simulink model "cartpole_pulse"  (R2024b)
settings: Solver=ode45  StartTime=0.0  StopTime=8  MaxStep=0.001  RelTol=1e-10  AbsTol=1e-12
model workspace (MAT data in the model file):
  A = [0  1  0  0; 0  -0.181818181818  2.67545454545  0; 0  0  0  1; 0  -0.454545454545  31.2136363636  0]
  B = [0; 1.81818181818; 0; 4.54545454545]
  K = [-38.7298334621 -36.3830062182 160.925764173 29.6787056292]
  pulse_amplitude = 2
  x0 = [0; 0; 0; 0]
Description:
  | Undergraduate thesis reimplementation. State=[x v theta omega], SI units; xc=x-l*sin(theta). Model Workspace contains exact Table 1 parameters and baseline A controller.
settings Model: ModifiedByFormat=WANG Zheng  Creator=WANG Zheng  LastModifiedBy=WANG Zheng
settings DataIOCC: OutputOption=SpecifiedOutputTimes  OutputTimes=[0:0.001:8]

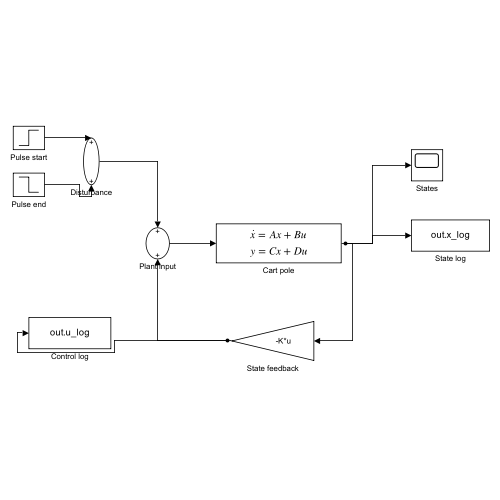
[thumbnail: Simulink's stored preview of the top-level diagram]
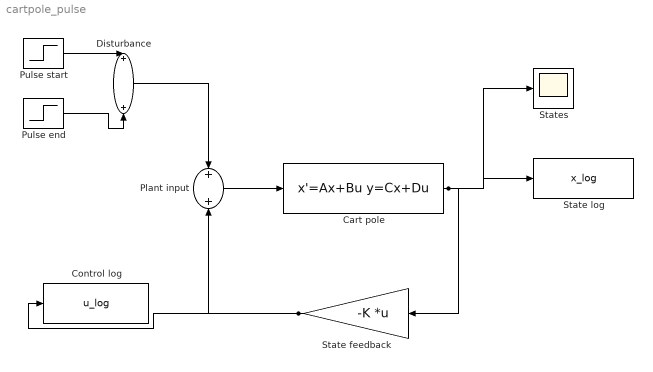
== system cartpole_pulse ==
  Cart pole : StateSpace  A=A  B=B  C=eye(4)  D=zeros(4,1)  InitialCondition=x0
  Control log : ToWorkspace  VariableName=u_log  SaveFormat=Timeseries  SampleTime=-1
  Disturbance : Sum
  Plant input : Sum
  Pulse end : Step  Time=1.2  After=-pulse_amplitude  SampleTime=0
  Pulse start : Step  After=pulse_amplitude  SampleTime=0
  State feedback : Gain  Gain=-K  Multiplication=Matrix(K*u)
  State log : ToWorkspace  VariableName=x_log  SaveFormat=Timeseries  SampleTime=-1
  States : Scope
  wires:
  Pulse start/1 -> Disturbance/1
  Pulse end/1 -> Disturbance/2
  Disturbance/1 -> Plant input/1
  State feedback/1 -> Plant input/2, Control log/1
  Plant input/1 -> Cart pole/1
  Cart pole/1 -> State feedback/1, State log/1, States/1
